simulink model "Lab0"  (R2024a)
settings: Solver=ode5  StartTime=0.0  StopTime=10  FixedStep=1e-03  RelTol=1e-3
undefined symbols (not defined in the file): Kd, Ki, Kp, mot, National_Instruments, PCI, sens, TL
libraries: sldrtlib x3
settings Model: SimulationMode=external  ExtModeTrigDuration=10000  Creator=lenovo  LastModifiedBy=lenovo
settings DataIOCC: ReturnWorkspaceOutputs=off
settings HardwareCC: ProdBitPerLong=64  ProdHWDeviceType=Intel->x86-64 (Linux 64)
settings RTWCC: Description=Simulink Desktop Real-Time  SystemTargetFile=sldrt.tlc  TemplateMakefile=sldrt.tmf  RTWCompilerOptimization=on
settings CodeAppCC: MaxIdLength=95
settings SimulinkDesktopRealTimeCC: TargetLibSuffix=_sldrt.a  TargetPreCompLibLocation=D:\Matlab2024\toolbox\sldrt\lib\win64

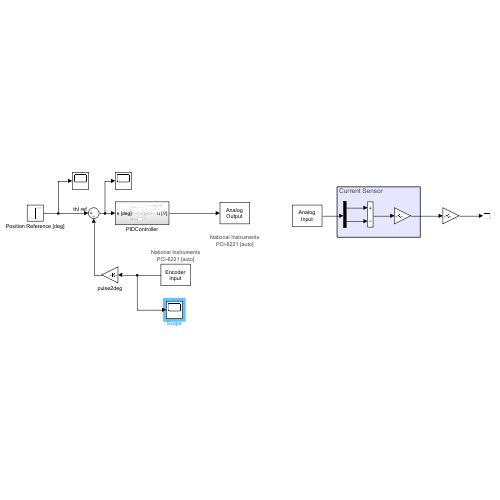
[thumbnail: Simulink's stored preview of the top-level diagram]
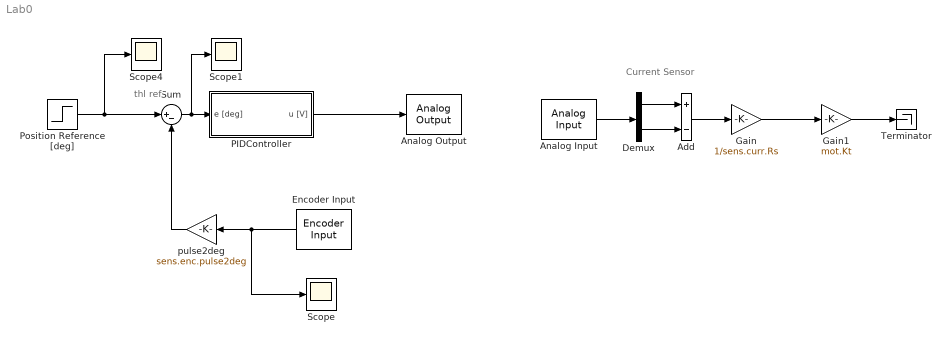
== system Lab0 ==
  note: Current Sensor
  note: thl ref
  Add : Sum  Inputs=+-
  Analog Input : sldrtlib/Analog Input  SampleTime=-1  MaxMissedTicks=10  ShowMissedTicks=off  YieldWhenWaiting=off  DrvAddress=0  DrvOptions=0  Channels=[1,2]  RangeMode=1  VoltRange=1  DataType=1
  Analog Output : sldrtlib/Analog Output  SampleTime=-1  MaxMissedTicks=10  ShowMissedTicks=off  YieldWhenWaiting=off  DrvName=National_Instruments/PCI-6221  DrvAddress=4294967295  DrvOptions=[0 0 0 2 0]  Channels=1  RangeMode=1  VoltRange=1  InitialValue=0  FinalValue=0
      settings: AttributesFormatString=National Instruments\nPCI-6221 [auto]
  Demux : Demux  Outputs=2
  Encoder Input : sldrtlib/Encoder Input  SampleTime=-1  MaxMissedTicks=10  ShowMissedTicks=off  YieldWhenWaiting=off  DrvName=National_Instruments/PCI-6221  DrvAddress=4294967295  DrvOptions=[0 0 0 2 0]  Channels=1  QuadMode=3  IndexPulse=1  InputFilter=Inf  DataType=1
      settings: AttributesFormatString=National Instruments\nPCI-6221 [auto]
  Gain : Gain  Gain=1/sens.curr.Rs
  Gain1 : Gain  Gain=mot.Kt
  PIDController : Subsystem
  Position Reference [deg] : Step  After=10  SampleTime=0
  Scope : Scope
  Scope1 : Scope
  Scope4 : Scope
  Sum : Sum  Inputs=|+-
  Terminator : Terminator
  pulse2deg : Gain  Gain=sens.enc.pulse2deg
  wires:
  Position Reference [deg]/1 -> Scope4/1, Sum/1
  Encoder Input/1 -> pulse2deg/1, Scope/1
  Sum/1 -> PIDController/1(e [deg]), Scope1/1
  PIDController/1(u [V]) -> Analog Output/1
  pulse2deg/1 -> Sum/2
  Gain/1 -> Gain1/1
  Demux/2 -> Add/2
  Analog Input/1 -> Demux/1
  Add/1 -> Gain/1
  Demux/1 -> Add/1
  Gain1/1 -> Terminator/1

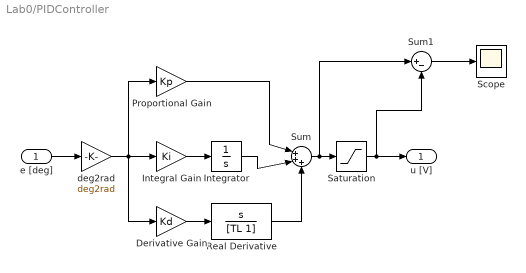
== system Lab0/PIDController ==
  e [deg] : Inport
  Derivative Gain : Gain  Gain=Kd
  Integral Gain : Gain  Gain=Ki
  Integrator : Integrator
  Proportional Gain : Gain  Gain=Kp
  Real Derivative : TransferFcn  Numerator=[1 0]  Denominator=[TL 1]
  Saturation : Saturate  UpperLimit=12  LowerLimit=-12
  Scope : Scope
  Sum : Sum  Inputs=|+++
  Sum1 : Sum  Inputs=|+-
  deg2rad : Gain  Gain=deg2rad
  u [V] : Outport
  wires:
  Saturation/1 -> Sum1/2, u [V]/1
  Sum/1 -> Sum1/1, Saturation/1
  Real Derivative/1 -> Sum/3
  Sum1/1 -> Scope/1
  Integral Gain/1 -> Integrator/1
  deg2rad/1 -> Derivative Gain/1, Proportional Gain/1, Integral Gain/1
  Integrator/1 -> Sum/2
  e [deg]/1 -> deg2rad/1
  Proportional Gain/1 -> Sum/1
  Derivative Gain/1 -> Real Derivative/1
